simulink model "vehical_behavior"  (R2025a)
settings: Solver=VariableStepAuto  StartTime=0.0  StopTime=10.0  RelTol=1e-3
settings Model: DataDictionary=vehicle_data.sldd  Creator=nikul  LastModifiedBy=nikul

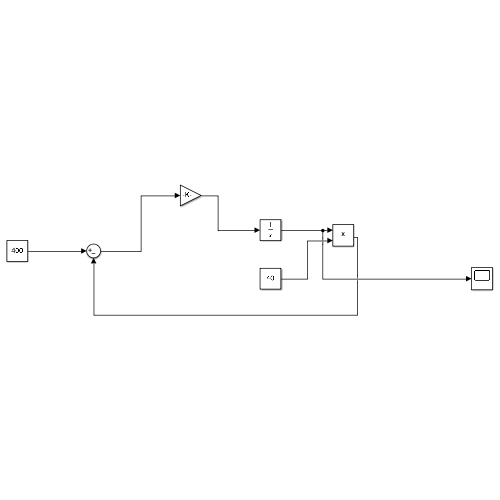
[thumbnail: Simulink's stored preview of the top-level diagram]
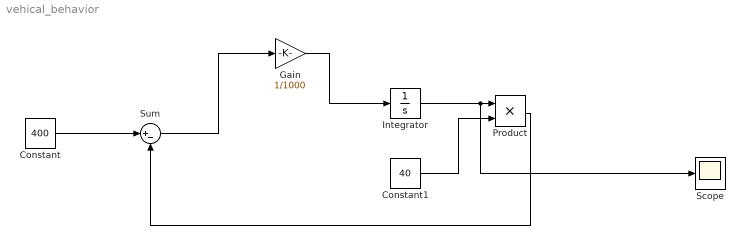
== system vehical_behavior ==
  Constant : Constant  Value=400
  Constant1 : Constant  Value=40
  Gain : Gain  Gain=1/1000
  Integrator : Integrator
  Product : Product
  Scope : Scope
      settings: ActiveDisplayYMinimum=-0.41209994245544784  ActiveDisplayYMaximum=3.7088994820990315
  Sum : Sum  Inputs=|+-
  wires:
  Constant/1 -> Sum/1
  Integrator/1 -> Scope/1, Product/1
  Product/1 -> Sum/2
  Sum/1 -> Gain/1
  Gain/1 -> Integrator/1
  Constant1/1 -> Product/2
